simulink model "btms_life_simulink"  (R2026b)
settings: Solver=FixedStepDiscrete  StopTime=simp.t_stop  FixedStep=simp.dt
InitFcn:
  | if ~(exist('P', 'var') && exist('cfg', 'var') && exist('simp', 'var'))
  |     addpath(fileparts(get_param(bdroot, 'FileName')));
  |     btms_sim_params(0);
  | end
values from neighbouring files (symbols this model uses):
  cfg = rmfield(c, 'name')    [btms_sim_params.m]    (also in run_simulink_validation.m = strategy_config(P, 'LIFE'))
  P = bms_params()    [btms_sim_params.m]    (also in run_simulink_validation.m)
  simp = struct('dt', 1, 'Ta', Ta, 'T0', Ta, 'SOH0', 1, 'soc_target', 0.80,      'x0', [Ta; Ta; 0.20; 0], 't_stop', 7200, 'T_heat', -1e9)    [btms_sim_params.m]
libraries: simulink x1
settings Model: Creator=karol  LastModifiedBy=karol
settings DataIOCC: SaveOutput=off  SaveTime=off  SignalLogging=off

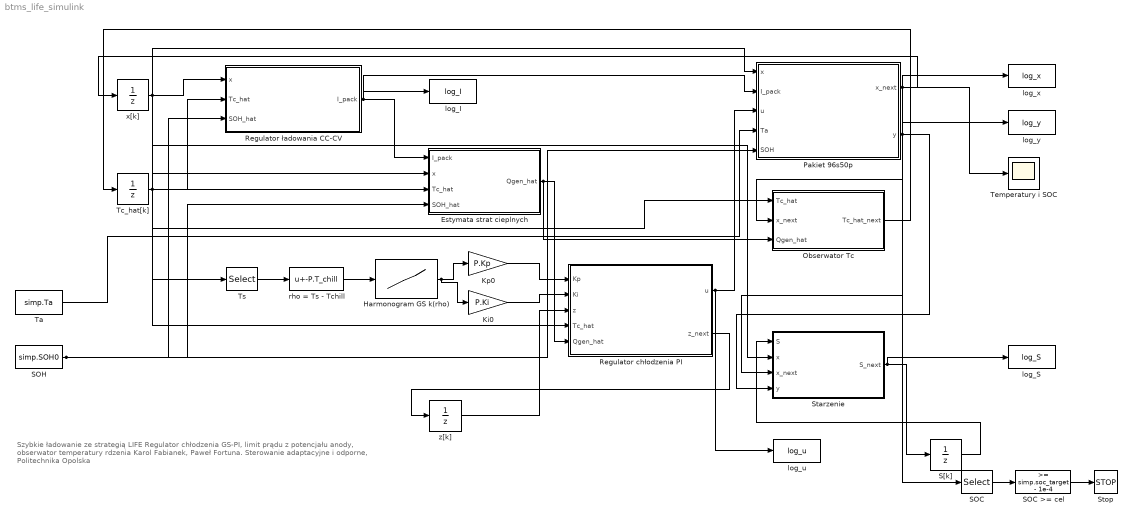
== system btms_life_simulink ==
  note: Szybkie ładowanie ze strategią LIFE
      | Regulator chłodzenia GS-PI, limit prądu z potencjału anody, obserwator temperatury rdzenia
      | Karol Fabianek, Paweł Fortuna. Sterowanie adaptacyjne i odporne, Politechnika Opolska
  Estymata strat cieplnych : MATLAB Function  TreatAsAtomicUnit=on
  Harmonogram GS k(rho) : Lookup_n-D  NumberOfTableDimensions=1  BreakpointsForDimension1=simp.gs_rho_bp  Table=simp.gs_k_tab  ExtrapMethod=Clip  InternalRulePriority=Speed  RndMeth=Simplest
  Ki0 : Gain  Gain=P.Ki
  Kp0 : Gain  Gain=P.Kp
  Obserwator Tc : MATLAB Function  TreatAsAtomicUnit=on
  Pakiet 96s50p : MATLAB Function  TreatAsAtomicUnit=on
  Regulator chłodzenia PI : MATLAB Function  TreatAsAtomicUnit=on
  Regulator ładowania CC-CV : MATLAB Function  TreatAsAtomicUnit=on
  SOC : Selector  InputPortWidth=4  IndexOptions=Index vector (dialog)  Indices=3  OutputSizes=1
  SOC >= cel : simulink/Logic and Bit Operations/Compare To Constant  relop=>=  const=simp.soc_target - 1e-4  OutDataTypeStr=boolean
  SOH : Constant  Value=simp.SOH0
  S[k] : UnitDelay  InitialCondition=[0; 0; 0]  SampleTime=simp.dt
  Starzenie : MATLAB Function  TreatAsAtomicUnit=on
  Stop : Stop
  Ta : Constant  Value=simp.Ta
  Tc_hat[k] : UnitDelay  InitialCondition=simp.T0  SampleTime=simp.dt
  Temperatury i SOC : Scope
  Ts : Selector  InputPortWidth=4  IndexOptions=Index vector (dialog)  Indices=2  OutputSizes=1
  log_I : ToWorkspace  VariableName=log_I  SampleTime=-1
  log_S : ToWorkspace  VariableName=log_S  SampleTime=-1
  log_u : ToWorkspace  VariableName=log_u  SampleTime=-1
  log_x : ToWorkspace  VariableName=log_x  SampleTime=-1
  log_y : ToWorkspace  VariableName=log_y  SampleTime=-1
  rho = Ts - Tchill : Bias  Bias=-P.T_chill  SaturateOnIntegerOverflow=off
  x[k] : UnitDelay  InitialCondition=simp.x0  SampleTime=simp.dt
  z[k] : UnitDelay  SampleTime=simp.dt
  wires:
  x[k]/1 -> Regulator ładowania CC-CV/1(x), Estymata strat cieplnych/2(x), Ts/1, Pakiet 96s50p/1(x), Starzenie/2(x)
  Tc_hat[k]/1 -> Regulator ładowania CC-CV/2(Tc_hat), Estymata strat cieplnych/3(Tc_hat), Regulator chłodzenia PI/4(Tc_hat), Obserwator Tc/1(Tc_hat)
  SOH/1 -> Regulator ładowania CC-CV/3(SOH_hat), Estymata strat cieplnych/4(SOH_hat), Pakiet 96s50p/5(SOH)
  Regulator ładowania CC-CV/1(I_pack) -> Estymata strat cieplnych/1(I_pack), Pakiet 96s50p/2(I_pack), log_I/1
  Ts/1 -> rho = Ts - Tchill/1
  rho = Ts - Tchill/1 -> Harmonogram GS k(rho)/1
  Harmonogram GS k(rho)/1 -> Kp0/1, Ki0/1
  Kp0/1 -> Regulator chłodzenia PI/1(Kp)
  Ki0/1 -> Regulator chłodzenia PI/2(Ki)
  z[k]/1 -> Regulator chłodzenia PI/3(z)
  Estymata strat cieplnych/1(Qgen_hat) -> Regulator chłodzenia PI/5(Qgen_hat), Obserwator Tc/3(Qgen_hat)
  Regulator chłodzenia PI/2(z_next) -> z[k]/1
  Regulator chłodzenia PI/1(u) -> Pakiet 96s50p/3(u), log_u/1
  Ta/1 -> Pakiet 96s50p/4(Ta)
  Pakiet 96s50p/1(x_next) -> x[k]/1, Obserwator Tc/2(x_next), Starzenie/3(x_next), SOC/1, log_x/1, Temperatury i SOC/1
  Obserwator Tc/1(Tc_hat_next) -> Tc_hat[k]/1
  S[k]/1 -> Starzenie/1(S)
  Pakiet 96s50p/2(y) -> Starzenie/4(y), log_y/1
  Starzenie/1(S_next) -> S[k]/1, log_S/1
  SOC/1 -> SOC >= cel/1
  SOC >= cel/1 -> Stop/1

== matlab function btms_life_simulink/Estymata strat cieplnych ==
  data: I_pack input; Qgen_hat output; x input; Tc_hat input; SOH_hat input; P parameter
function Qgen_hat = fcn(I_pack, x, Tc_hat, SOH_hat, P)
[R0, R1] = cell_resistance(P, Tc_hat, x(3), SOH_hat);
Qgen_hat = P.ns*P.np*(I_pack/P.np)^2*(R0 + R1);

== matlab function btms_life_simulink/Regulator ładowania CC-CV ==
  data: x input; I_pack output; Tc_hat input; SOH_hat input; P parameter; cfg parameter; simp parameter
function I_pack = fcn(x, Tc_hat, SOH_hat, P, cfg, simp)
% Warstwowy limit prądu: CC-CV, nadzór termiczny, potencjał anody
I_pack = charge_controller(P, cfg, true, x(3), simp.soc_target, Tc_hat, x(4), SOH_hat, simp.dt);

== matlab function btms_life_simulink/Regulator chłodzenia PI ==
  data: Kp input; u output; Ki input; z input; Tc_hat input; Qgen_hat input; z_next output; P parameter; cfg parameter; simp parameter
function [u, z_next] = fcn(Kp, Ki, z, Tc_hat, Qgen_hat, P, cfg, simp)
% Działanie odwrotne, anti-windup przez całkowanie warunkowe
if Tc_hat < simp.T_heat
    u = -min(1, P.Kh*(simp.T_heat - Tc_hat)); z_next = 0; return
end
e = Tc_hat - P.Tref_charge;
FF = cfg.ff*P.ff_gain*Qgen_hat/P.Qcool_max;
u_raw = Kp*e + z + FF;
u = min(1, max(0, u_raw));
if (u_raw >= 1 && e > 0) || (u_raw <= 0 && e < 0)
    z_next = z;
else
    z_next = z + Ki*simp.dt*e;
end

== matlab function btms_life_simulink/Pakiet 96s50p ==
  data: x input; I_pack input; x_next output; u input; y output; Ta input; SOH input; P parameter; simp parameter
function [x_next, y] = fcn(x, I_pack, u, Ta, SOH, P, simp)
[x_next, y] = pack_step(P, x, I_pack, u, Ta, simp.dt, SOH);

== matlab function btms_life_simulink/Obserwator Tc ==
  data: Tc_hat input; Tc_hat_next output; x_next input; Qgen_hat input; P parameter; simp parameter
function Tc_hat_next = fcn(Tc_hat, x_next, Qgen_hat, P, simp)
Tc_hat_next = core_observer(P, Tc_hat, x_next(2), Qgen_hat, simp.dt);

== matlab function btms_life_simulink/Starzenie ==
  data: S input; S_next output; x input; x_next input; y input; P parameter; simp parameter
function S_next = fcn(S, x, x_next, y, P, simp)
s = aging_stress(P, 0.5*(x(1) + x_next(1)), x(3), y(6), y(7), simp.dt);
S_next = S(:) + s(:);
